simulink model "nadir_pid_testbench"  (R2025a)
settings: Solver=ode4  StartTime=0.0  StopTime=tStop  FixedStep=dt  RelTol=1e-3
model workspace (MAT data in the model file):
  AOCS.Spacecraft.I_B = [0.0409  0  0; 0  0.0403  0; 0  0  0.0073]
  AOCS.GNC.SampleTime_s = 0.1
  AOCS.Control.PIDKp_s2 = 0.003924
  AOCS.Control.PIDKd_s = 0.14625
  AOCS.Control.Ki_s3 = 8.1e-06
  AOCS.Control.AntiWindupTime_s = 150
  AOCS.Control.MaxTorque_Nm = 2e-05
  AOCS.Control.Enabled = 1
  AOCS.Control.UseIntegral = 1
  J = [0.0409  0  0; 0  0.0403  0; 0  0  0.0073]
  Ts = 0.1
  dt = 0.01
  omega0 = [0; 0; 0]
  q0 = [0.999048221582; 0.0436193873653; 0; 0]
  q_ref = [1; 0; 0; 0]
  tStop = 600
  tau_ext = [0; 0; 0]
libraries: aerolibutil x4, sharedutil x4, matrix_library x2
Description:
  | Unmodified production PID connected to a simple rigid body. Parameters saved in Model Workspace; no setup.
settings Model: Creator=juliankazmierski  LastModifiedBy=juliankazmierski
settings DataIOCC: SaveOutput=off

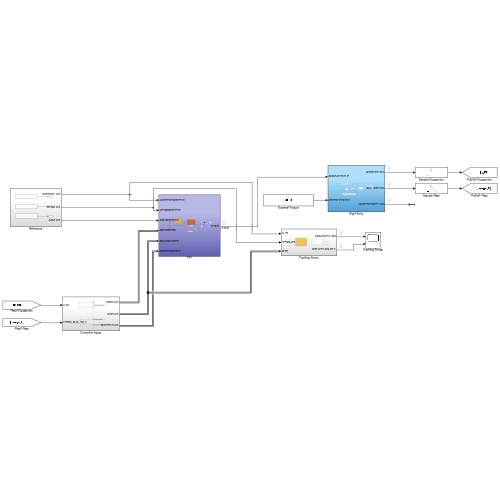
[thumbnail: Simulink's stored preview of the top-level diagram]
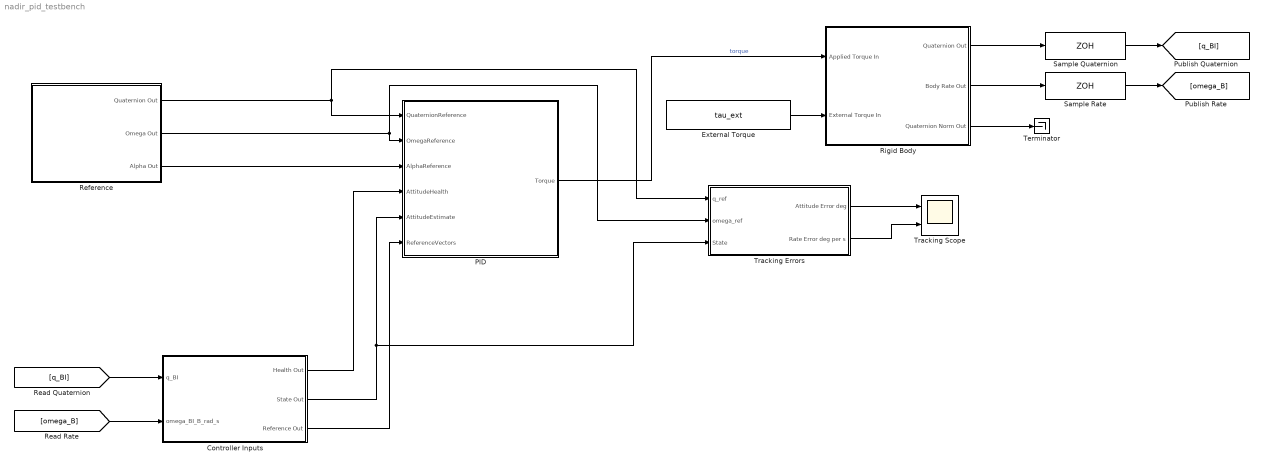
== system nadir_pid_testbench ==
  Controller Inputs : Subsystem
  External Torque : Constant  Value=tau_ext  VectorParams1D=off
  PID : Subsystem  Description=|
      | Copy of PD with integral feedback on 2*q_error(2:4).
      | xi_dot = Ki*e_theta - J^(-1)*(tau_sat-tau_demand)/Taw; u_PID = u_PD-xi.
      | Forward Euler at the GNC tick; reset when inactive. No external torque input.
  Reference : Subsystem
  Rigid Body : Subsystem
  Sample Quaternion : ZeroOrderHold  SampleTime=Ts
  Sample Rate : ZeroOrderHold  SampleTime=Ts
  Terminator : Terminator
  Tracking Errors : Subsystem
  Tracking Scope : Scope  NumInputPorts=2
      settings: TimeSpan=600  ActiveDisplayYMinimum=-0.56906498733131183  ActiveDisplayYMaximum=0.88179362660269689
  wires:
  [q_BI] -> Controller Inputs/1(q_BI)
  [omega_B] -> Controller Inputs/2(omega_BI_B_rad_s)
  Controller Inputs/1(Health Out) -> PID/4(AttitudeHealth)
  Reference/1(Quaternion Out) -> PID/1(QuaternionReference), Tracking Errors/1(q_ref)
  Controller Inputs/2(State Out) -> Tracking Errors/3(State), PID/5(AttitudeEstimate)
  Reference/2(Omega Out) -> PID/2(OmegaReference), Tracking Errors/2(omega_ref)
  Controller Inputs/3(Reference Out) -> PID/6(ReferenceVectors)
  Reference/3(Alpha Out) -> PID/3(AlphaReference)
  PID/1(Torque) -> Rigid Body/1(Applied Torque In)  "torque"
  External Torque/1 -> Rigid Body/2(External Torque In)
  Rigid Body/1(Quaternion Out) -> Sample Quaternion/1
  Sample Quaternion/1 -> [q_BI]
  Rigid Body/2(Body Rate Out) -> Sample Rate/1
  Sample Rate/1 -> [omega_B]
  Rigid Body/3(Quaternion Norm Out) -> Terminator/1
  Tracking Errors/1(Attitude Error deg) -> Tracking Scope/1
  Tracking Errors/2(Rate Error deg per s) -> Tracking Scope/2

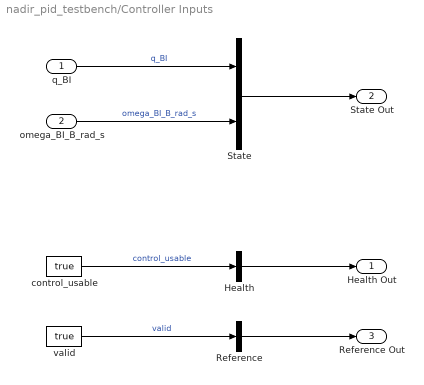
== system nadir_pid_testbench/Controller Inputs ==
  q_BI : Inport
  omega_BI_B_rad_s : Inport  Port=2
  Health : BusCreator  Inputs=1
  Reference : BusCreator  Inputs=1
  State : BusCreator  Inputs=2
  control_usable : Constant  Value=true  OutDataTypeStr=boolean
  valid : Constant  Value=true  OutDataTypeStr=boolean
  Health Out : Outport
  State Out : Outport  Port=2
  Reference Out : Outport  Port=3
  wires:
  q_BI/1 -> State/1  "q_BI"
  omega_BI_B_rad_s/1 -> State/2  "omega_BI_B_rad_s"
  control_usable/1 -> Health/1  "control_usable"
  valid/1 -> Reference/1  "valid"
  Health/1 -> Health Out/1
  State/1 -> State Out/1
  Reference/1 -> Reference Out/1

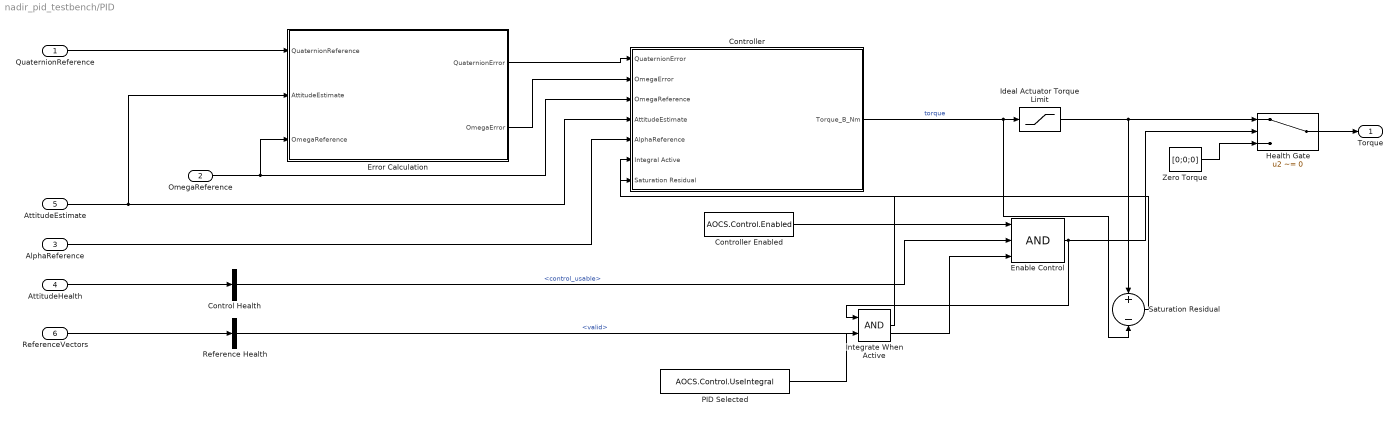
== system nadir_pid_testbench/PID ==
  QuaternionReference : Inport
  OmegaReference : Inport  Port=2
  AlphaReference : Inport  Port=3
  AttitudeHealth : Inport  Port=4
  AttitudeEstimate : Inport  Port=5
  ReferenceVectors : Inport  Port=6
  Control Health : BusSelector  OutputSignals=control_usable
  Controller : Subsystem  Description=|
      | Quaternion PD with rigid-body dynamic compensation.
      | qe scalar-first, C_BD maps desired D components into body B.
      | eOmega = omegaHat - C_BD*omegaRef_D.
      | tau = omegaHat x (J*omegaHat) + J*(-2*Kp*qe_v-Kd*eOmega-eOmega x (C_BD*omegaRef_D)+C_BD*alphaRef_D).
      | Gains have units 1/s^2 and 1/s. This cancels rate dynamics, not quaternion kinematics.
  Controller Enabled : Constant  Value=AOCS.Control.Enabled  OutDataTypeStr=boolean
  Enable Control : Logic  Inputs=3  AllPortsSameDT=off  OutDataTypeStr=boolean
  Error Calculation : Subsystem
  Health Gate : Switch  Criteria=u2 ~= 0  SaturateOnIntegerOverflow=off  InputSameDT=off
  Ideal Actuator Torque Limit : Saturate  UpperLimit=AOCS.Control.MaxTorque_Nm  LowerLimit=-AOCS.Control.MaxTorque_Nm
  Integrate When Active : Logic  AllPortsSameDT=off  OutDataTypeStr=boolean
  PID Selected : Constant  Value=AOCS.Control.UseIntegral  OutDataTypeStr=boolean
  Reference Health : BusSelector  OutputSignals=valid
  Saturation Residual : Sum  Inputs=+-
  Zero Torque : Constant  Value=[0;0;0]  VectorParams1D=off
  Torque : Outport
  wires:
  Saturation Residual/1 -> Controller/7(Saturation Residual)
  Integrate When Active/1 -> Controller/6(Integral Active)
  PID Selected/1 -> Integrate When Active/2
  AttitudeEstimate/1 -> Controller/4(AttitudeEstimate), Error Calculation/2(AttitudeEstimate)
  Error Calculation/2(OmegaError) -> Controller/2(OmegaError)
  OmegaReference/1 -> Controller/3(OmegaReference), Error Calculation/3(OmegaReference)
  Enable Control/1 -> Integrate When Active/1, Health Gate/2
  Error Calculation/1(QuaternionError) -> Controller/1(QuaternionError)
  Control Health/1 -> Enable Control/2  "<control_usable>"
  QuaternionReference/1 -> Error Calculation/1(QuaternionReference)
  AttitudeHealth/1 -> Control Health/1
  Controller Enabled/1 -> Enable Control/1
  ReferenceVectors/1 -> Reference Health/1
  AlphaReference/1 -> Controller/5(AlphaReference)
  Controller/1(Torque_B_Nm) -> Saturation Residual/2, Ideal Actuator Torque Limit/1  "torque"
  Health Gate/1 -> Torque/1
  Reference Health/1 -> Enable Control/3  "<valid>"
  Ideal Actuator Torque Limit/1 -> Saturation Residual/1, Health Gate/1
  Zero Torque/1 -> Health Gate/3

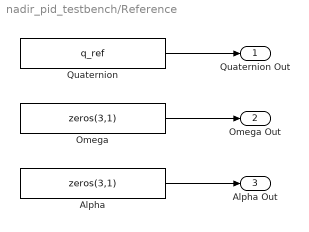
== system nadir_pid_testbench/Reference ==
  Alpha : Constant  Value=zeros(3,1)  VectorParams1D=off
  Omega : Constant  Value=zeros(3,1)  VectorParams1D=off
  Quaternion : Constant  Value=q_ref  VectorParams1D=off
  Quaternion Out : Outport
  Omega Out : Outport  Port=2
  Alpha Out : Outport  Port=3
  wires:
  Quaternion/1 -> Quaternion Out/1
  Omega/1 -> Omega Out/1
  Alpha/1 -> Alpha Out/1

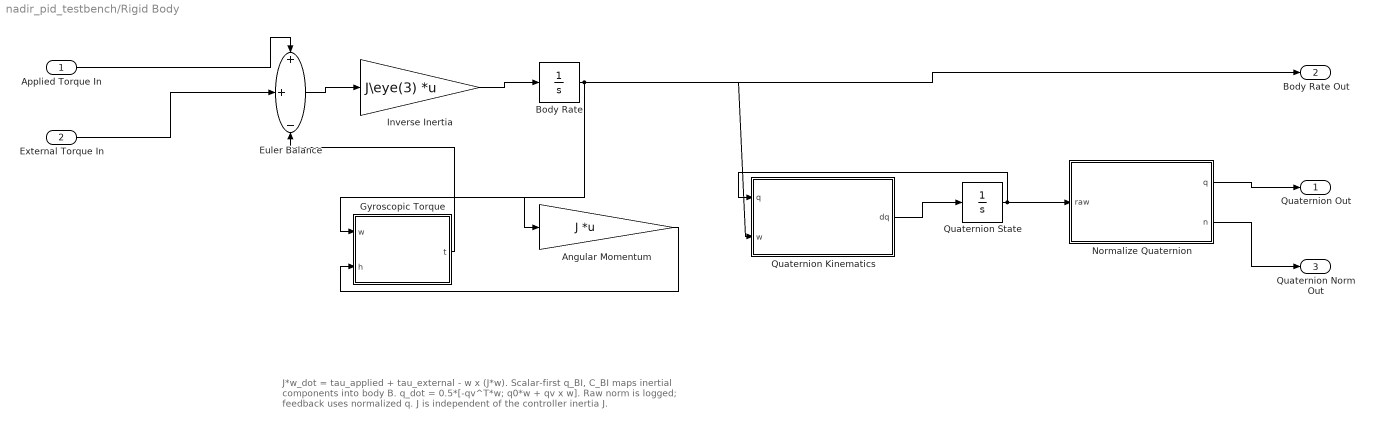
== system nadir_pid_testbench/Rigid Body ==
  note: J*w_dot = tau_applied + tau_external - w x (J*w).
      | Scalar-first q_BI, C_BI maps inertial components into body B.
      | q_dot = 0.5*[-qv^T*w; q0*w + qv x w]. Raw norm is logged; feedback uses normalized q.
      | J is independent of the controller inertia J.
  Applied Torque In : Inport
  External Torque In : Inport  Port=2
  Angular Momentum : Gain  Gain=J  Multiplication=Matrix(K*u)
  Body Rate : Integrator  InitialCondition=omega0
  Euler Balance : Sum  Inputs=++-
  Gyroscopic Torque : MATLAB Function  TreatAsAtomicUnit=on
  Inverse Inertia : Gain  Gain=J\eye(3)  Multiplication=Matrix(K*u)
  Normalize Quaternion : MATLAB Function  TreatAsAtomicUnit=on
  Quaternion Kinematics : MATLAB Function  TreatAsAtomicUnit=on
  Quaternion State : Integrator  InitialCondition=q0/norm(q0)
  Quaternion Out : Outport
  Body Rate Out : Outport  Port=2
  Quaternion Norm Out : Outport  Port=3
  wires:
  Applied Torque In/1 -> Euler Balance/1
  External Torque In/1 -> Euler Balance/2
  Gyroscopic Torque/1(t) -> Euler Balance/3
  Euler Balance/1 -> Inverse Inertia/1
  Inverse Inertia/1 -> Body Rate/1
  Body Rate/1 -> Angular Momentum/1, Gyroscopic Torque/1(w), Quaternion Kinematics/2(w), Body Rate Out/1
  Angular Momentum/1 -> Gyroscopic Torque/2(h)
  Quaternion State/1 -> Quaternion Kinematics/1(q), Normalize Quaternion/1(raw)
  Quaternion Kinematics/1(dq) -> Quaternion State/1
  Normalize Quaternion/1(q) -> Quaternion Out/1
  Normalize Quaternion/2(n) -> Quaternion Norm Out/1

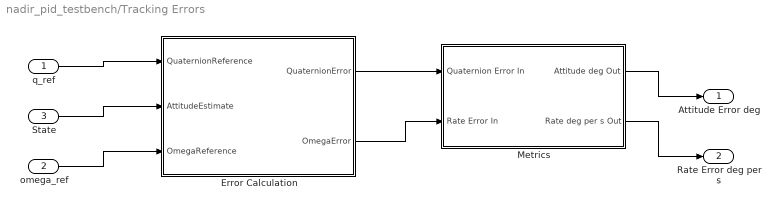
== system nadir_pid_testbench/Tracking Errors ==
  q_ref : Inport
  omega_ref : Inport  Port=2
  State : Inport  Port=3
  Error Calculation : Subsystem
  Metrics : Subsystem
  Attitude Error deg : Outport
  Rate Error deg per s : Outport  Port=2
  wires:
  q_ref/1 -> Error Calculation/1(QuaternionReference)
  State/1 -> Error Calculation/2(AttitudeEstimate)
  omega_ref/1 -> Error Calculation/3(OmegaReference)
  Error Calculation/1(QuaternionError) -> Metrics/1(Quaternion Error In)
  Metrics/1(Attitude deg Out) -> Attitude Error deg/1
  Error Calculation/2(OmegaError) -> Metrics/2(Rate Error In)
  Metrics/2(Rate deg per s Out) -> Rate Error deg per s/1

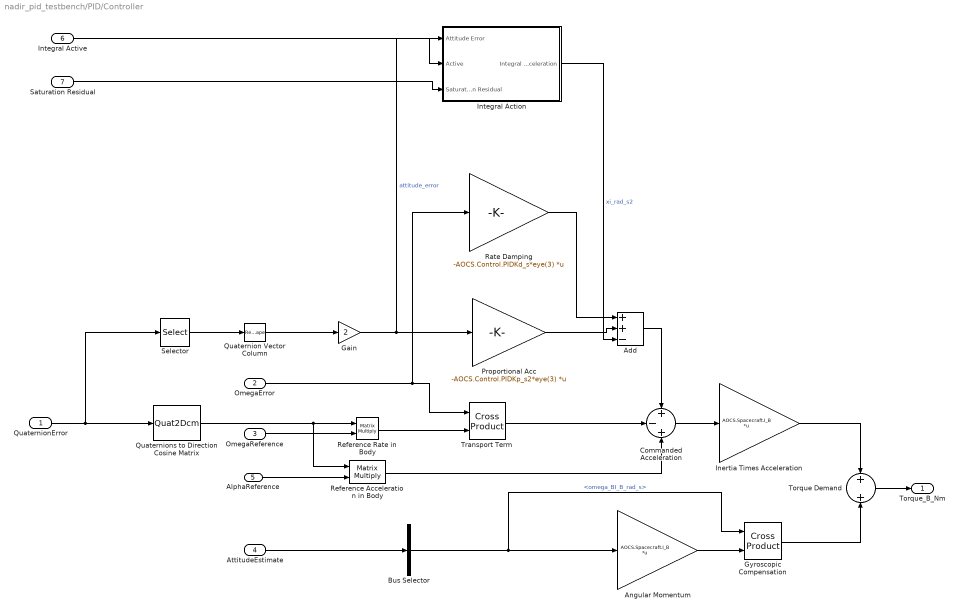
== system nadir_pid_testbench/PID/Controller ==
  QuaternionError : Inport
  OmegaError : Inport  Port=2
  OmegaReference : Inport  Port=3
  AttitudeEstimate : Inport  Port=4
  AlphaReference : Inport  Port=5
  Integral Active : Inport  Port=6
  Saturation Residual : Inport  Port=7
  Add : Sum  Inputs=++-
  Angular Momentum : Gain  Gain=AOCS.Spacecraft.I_B  Multiplication=Matrix(K*u)
  Bus Selector : BusSelector  OutputSignals=omega_BI_B_rad_s
  Commanded Acceleration : Sum  Inputs=+-+
  Gain : Gain  Gain=2
  Gyroscopic Compensation : matrix_library/Cross Product
  Inertia Times Acceleration : Gain  Gain=AOCS.Spacecraft.I_B  Multiplication=Matrix(K*u)
  Integral Action : Subsystem
  Proportional Acc : Gain  Gain=-AOCS.Control.PIDKp_s2*eye(3)  Multiplication=Matrix(K*u)
  Quaternion Vector Column : Reshape  OutputDimensionality=Customize  OutputDimensions=[3,1]
  Quaternions to Direction Cosine Matrix : Quat2Dcm
  Rate Damping : Gain  Gain=-AOCS.Control.PIDKd_s*eye(3)  Multiplication=Matrix(K*u)
  Reference Acceleration in Body : Product  Inputs=**  Multiplication=Matrix(*)
  Reference Rate in Body : Product  Multiplication=Matrix(*)
  Selector : Selector  InputPortWidth=4  IndexOptions=Index vector (dialog)  Indices=[2 3 4]  OutputSizes=1
  Torque Demand : Sum
  Transport Term : matrix_library/Cross Product
  Torque_B_Nm : Outport  PortDimensions=[3 1]
  wires:
  Integral Action/1(Integral Acceleration) -> Add/3  "xi_rad_s2"
  Saturation Residual/1 -> Integral Action/3(Saturation Residual)
  Integral Active/1 -> Integral Action/2(Active)
  Gyroscopic Compensation/1 -> Torque Demand/2
  QuaternionError/1 -> Selector/1, Quaternions to Direction Cosine Matrix/1
  Proportional Acc/1 -> Add/2
  Selector/1 -> Quaternion Vector Column/1
  Commanded Acceleration/1 -> Inertia Times Acceleration/1
  Torque Demand/1 -> Torque_B_Nm/1
  OmegaError/1 -> Rate Damping/1, Transport Term/1
  Quaternion Vector Column/1 -> Gain/1
  Inertia Times Acceleration/1 -> Torque Demand/1
  OmegaReference/1 -> Reference Rate in Body/2
  Angular Momentum/1 -> Gyroscopic Compensation/2
  Quaternions to Direction Cosine Matrix/1 -> Reference Rate in Body/1, Reference Acceleration in Body/1
  AttitudeEstimate/1 -> Bus Selector/1
  AlphaReference/1 -> Reference Acceleration in Body/2
  Reference Rate in Body/1 -> Transport Term/2
  Reference Acceleration in Body/1 -> Commanded Acceleration/3
  Gain/1 -> Integral Action/1(Attitude Error), Proportional Acc/1  "attitude_error"
  Rate Damping/1 -> Add/1
  Transport Term/1 -> Commanded Acceleration/2
  Add/1 -> Commanded Acceleration/1
  Bus Selector/1 -> Gyroscopic Compensation/1, Angular Momentum/1  "<omega_BI_B_rad_s>"

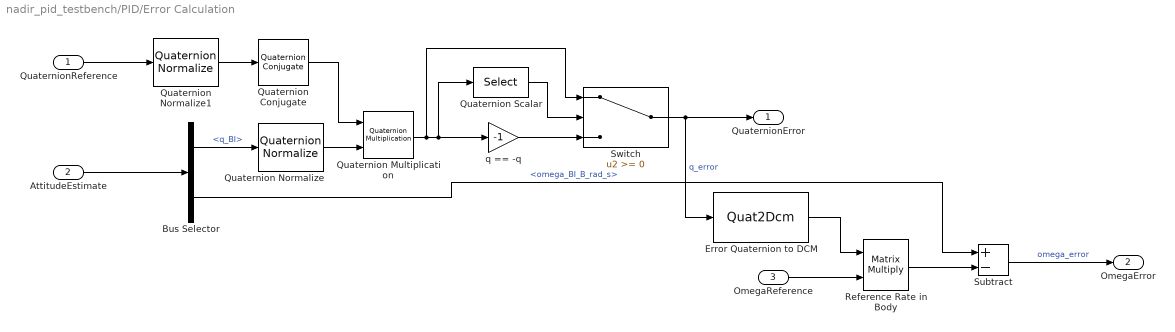
== system nadir_pid_testbench/PID/Error Calculation ==
  QuaternionReference : Inport
  AttitudeEstimate : Inport  Port=2
  OmegaReference : Inport  Port=3
  Bus Selector : BusSelector  OutputSignals=q_BI,omega_BI_B_rad_s
  Error Quaternion to DCM : Quat2Dcm
  Quaternion Conjugate : aerolibutil/Quaternion Conjugate
  Quaternion Multiplication : aerolibutil/Quaternion Multiplication
  Quaternion Normalize : sharedutil/Quaternion Normalize  aMode=aMode
  Quaternion Normalize1 : sharedutil/Quaternion Normalize  aMode=aMode
  Quaternion Scalar : Selector  InputPortWidth=4  IndexOptions=Index vector (dialog)  Indices=1  OutputSizes=1
  Reference Rate in Body : Product  Inputs=**  Multiplication=Matrix(*)
  Subtract : Sum  Inputs=+-
  Switch : Switch  SaturateOnIntegerOverflow=off  InputSameDT=off
  q == -q : Gain  Gain=-1
  QuaternionError : Outport
  OmegaError : Outport  Port=2
  wires:
  QuaternionReference/1 -> Quaternion Normalize1/1
  Quaternion Conjugate/1 -> Quaternion Multiplication/1
  AttitudeEstimate/1 -> Bus Selector/1
  Subtract/1 -> OmegaError/1  "omega_error"
  Quaternion Normalize/1 -> Quaternion Multiplication/2
  Quaternion Normalize1/1 -> Quaternion Conjugate/1
  Bus Selector/2 -> Subtract/1  "<omega_BI_B_rad_s>"
  Switch/1 -> QuaternionError/1, Error Quaternion to DCM/1  "q_error"
  Bus Selector/1 -> Quaternion Normalize/1  "<q_BI>"
  Quaternion Multiplication/1 -> Switch/1, Quaternion Scalar/1, q == -q/1
  Quaternion Scalar/1 -> Switch/2
  q == -q/1 -> Switch/3
  Error Quaternion to DCM/1 -> Reference Rate in Body/1
  OmegaReference/1 -> Reference Rate in Body/2
  Reference Rate in Body/1 -> Subtract/2

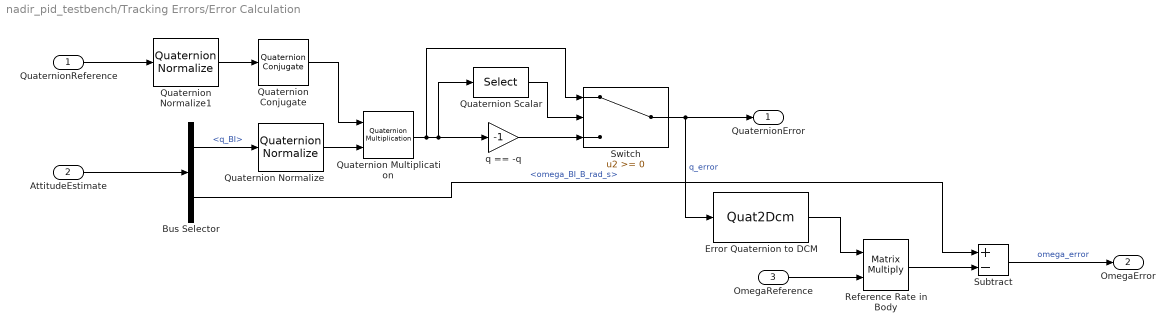
== system nadir_pid_testbench/Tracking Errors/Error Calculation ==
  QuaternionReference : Inport
  AttitudeEstimate : Inport  Port=2
  OmegaReference : Inport  Port=3
  Bus Selector : BusSelector  OutputSignals=q_BI,omega_BI_B_rad_s
  Error Quaternion to DCM : Quat2Dcm
  Quaternion Conjugate : aerolibutil/Quaternion Conjugate
  Quaternion Multiplication : aerolibutil/Quaternion Multiplication
  Quaternion Normalize : sharedutil/Quaternion Normalize  aMode=aMode
  Quaternion Normalize1 : sharedutil/Quaternion Normalize  aMode=aMode
  Quaternion Scalar : Selector  InputPortWidth=4  IndexOptions=Index vector (dialog)  Indices=1  OutputSizes=1
  Reference Rate in Body : Product  Inputs=**  Multiplication=Matrix(*)
  Subtract : Sum  Inputs=+-
  Switch : Switch  SaturateOnIntegerOverflow=off  InputSameDT=off
  q == -q : Gain  Gain=-1
  QuaternionError : Outport
  OmegaError : Outport  Port=2
  wires:
  Reference Rate in Body/1 -> Subtract/2
  OmegaReference/1 -> Reference Rate in Body/2
  Error Quaternion to DCM/1 -> Reference Rate in Body/1
  q == -q/1 -> Switch/3
  Quaternion Scalar/1 -> Switch/2
  Quaternion Multiplication/1 -> q == -q/1, Quaternion Scalar/1, Switch/1
  Bus Selector/1 -> Quaternion Normalize/1  "<q_BI>"
  Switch/1 -> Error Quaternion to DCM/1, QuaternionError/1  "q_error"
  Bus Selector/2 -> Subtract/1  "<omega_BI_B_rad_s>"
  Quaternion Normalize1/1 -> Quaternion Conjugate/1
  Quaternion Normalize/1 -> Quaternion Multiplication/2
  Subtract/1 -> OmegaError/1  "omega_error"
  AttitudeEstimate/1 -> Bus Selector/1
  Quaternion Conjugate/1 -> Quaternion Multiplication/1
  QuaternionReference/1 -> Quaternion Normalize1/1

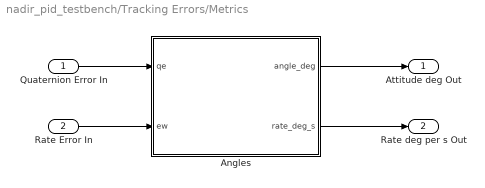
== system nadir_pid_testbench/Tracking Errors/Metrics ==
  Quaternion Error In : Inport
  Rate Error In : Inport  Port=2
  Angles : MATLAB Function  TreatAsAtomicUnit=on
  Attitude deg Out : Outport
  Rate deg per s Out : Outport  Port=2
  wires:
  Quaternion Error In/1 -> Angles/1(qe)
  Rate Error In/1 -> Angles/2(ew)
  Angles/1(angle_deg) -> Attitude deg Out/1
  Angles/2(rate_deg_s) -> Rate deg per s Out/1

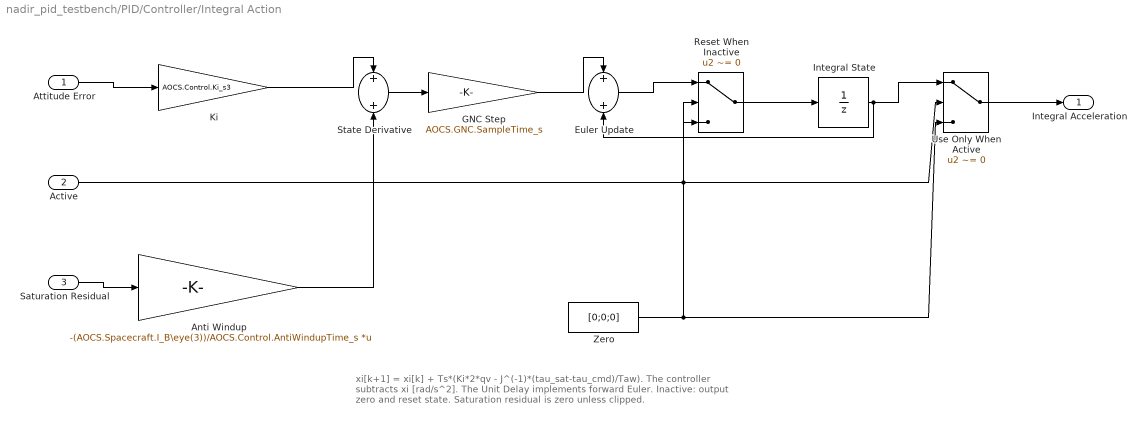
== system nadir_pid_testbench/PID/Controller/Integral Action ==
  note: xi[k+1] = xi[k] + Ts*(Ki*2*qv - J^(-1)*(tau_sat-tau_cmd)/Taw).
      | The controller subtracts xi [rad/s^2]. The Unit Delay implements forward Euler.
      | Inactive: output zero and reset state. Saturation residual is zero unless clipped.
  Attitude Error : Inport
  Active : Inport  Port=2
  Saturation Residual : Inport  Port=3
  Anti Windup : Gain  Gain=-(AOCS.Spacecraft.I_B\eye(3))/AOCS.Control.AntiWindupTime_s  Multiplication=Matrix(K*u)
  Euler Update : Sum
  GNC Step : Gain  Gain=AOCS.GNC.SampleTime_s
  Integral State : UnitDelay  InitialCondition=[0;0;0]  SampleTime=-1  HasFrameUpgradeWarning=on
  Ki : Gain  Gain=AOCS.Control.Ki_s3
  Reset When Inactive : Switch  Criteria=u2 ~= 0  SaturateOnIntegerOverflow=off  InputSameDT=off
  State Derivative : Sum
  Use Only When Active : Switch  Criteria=u2 ~= 0  SaturateOnIntegerOverflow=off  InputSameDT=off
  Zero : Constant  Value=[0;0;0]  VectorParams1D=off
  Integral Acceleration : Outport
  wires:
  Use Only When Active/1 -> Integral Acceleration/1
  Reset When Inactive/1 -> Integral State/1
  Zero/1 -> Use Only When Active/3, Reset When Inactive/3
  Active/1 -> Use Only When Active/2, Reset When Inactive/2
  Euler Update/1 -> Reset When Inactive/1
  Integral State/1 -> Use Only When Active/1, Euler Update/2
  GNC Step/1 -> Euler Update/1
  State Derivative/1 -> GNC Step/1
  Anti Windup/1 -> State Derivative/2
  Saturation Residual/1 -> Anti Windup/1
  Ki/1 -> State Derivative/1
  Attitude Error/1 -> Ki/1

== matlab function nadir_pid_testbench/Rigid Body/Gyroscopic Torque ==
  data: w input; t output; h input
function t = f(w,h)
t=cross(w,h);
end

== matlab function nadir_pid_testbench/Rigid Body/Normalize Quaternion ==
  data: raw input; q output; n output
function [q,n] = f(raw)
n=norm(raw); q=raw/n;
end

== matlab function nadir_pid_testbench/Tracking Errors/Metrics/Angles ==
  data: qe input; angle_deg output; ew input; rate_deg_s output
function [angle_deg, rate_deg_s] = f(qe,ew)
angle_deg=2*atan2(norm(qe(2:4)),abs(qe(1)))*180/pi;
rate_deg_s=norm(ew)*180/pi;
end

== matlab function nadir_pid_testbench/Rigid Body/Quaternion Kinematics ==
  data: q input; dq output; w input
function dq = f(q,w)
dq=0.5*[-q(2:4)'*w; q(1)*w+cross(q(2:4),w)];
end
